simulink subsystem "DABSecondaryMOSFETDevice"  (R2026a)
settings: Solver=VariableStepAuto
libraries: ConverterLibrary x1
settings Model: Creator=vsolaise  LastModifiedBy=vsolaise

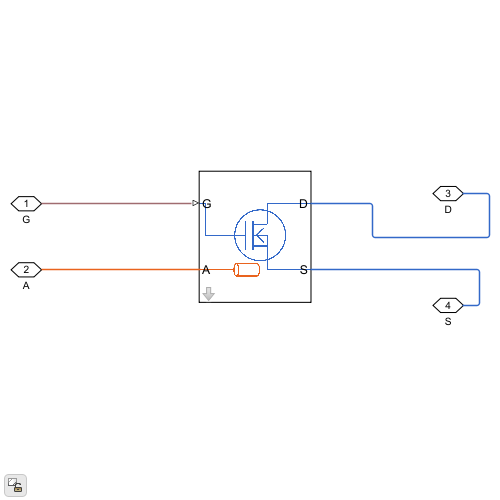
[thumbnail: Simulink's stored preview of the top-level diagram]
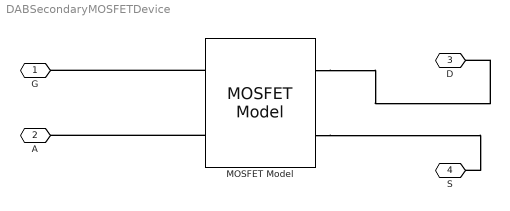
== system DABSecondaryMOSFETDevice ==
  MOSFET Model : ConverterLibrary/Components/MOSFET Model  Vth=DAB.SwitchSec.Vth V  Von_data=DAB.SwitchSec.Von_data V  Tj=DAB.SwitchSec.Tj degC  Iout_data=DAB.SwitchSec.Iout_data A  Iout_data_loss=DAB.SwitchSec.Iout_data_loss A  Tj_loss=DAB.SwitchSec.Tj_loss degC  Eoff_data=DAB.SwitchSec.Eoff_data J  Eon_data=DAB.SwitchSec.Eon_data J  Voff=DAB.SwitchSec.Voff V  Soft_Switching_Flag=on  Tj_diode=DAB.SwitchSec.diode_TjVec degC  If_data=DAB.SwitchSec.diode_IfVec A  Vf_data=DAB.SwitchSec.diode_VfMat V  thermal_resistance=DAB.SwitchSec.R K/W  thermal_mass=DAB.SwitchSec.junction_thermal_mass J/K  Tj0=DAB.simTempSec degC  Goff=DAB.SwitchSec.diode_Goff S  Rds=DAB.SwitchSec.Rds Ohm  GdsOff=DAB.SwitchSec.Goff S
      settings: SourceProductName=Simscape Power Converter Components
  G : PMIOPort  Side=Left
  A : PMIOPort  Port=2  Side=Left
  D : PMIOPort  Port=3  Side=Right
  S : PMIOPort  Port=4  Side=Right
  connections:
  MOSFET Model/LConn2 -- A/RConn1
  MOSFET Model/LConn1 -- G/RConn1
  MOSFET Model/RConn1 -- D/RConn1
  MOSFET Model/RConn2 -- S/RConn1
